simulink model "PSO_PI_Controlled_Booster"  (R2024a)
settings: Solver=VariableStepAuto  StartTime=0.0  StopTime=.2  RelTol=1e-3
values from neighbouring files (symbols this model uses):
  C = 470e-6    (= 0.00047)    [RLC_finder.m]
  Ki = Ki_all(ord(1))    [Run_PI_Optimization.m]    (also in Run_PI_Optimization_paper.m)
  Kp = Kp_all(ord(1))    [Run_PI_Optimization.m]    (also in Run_PI_Optimization_paper.m)
  L = 22.5e-6    (= 2.25e-05)    [RLC_finder.m]    (also in Run_HW_Retest.m = splitlines(string(buf(1:k))))
  R = [2.14277391959 2.34771272008 1.46812094374 4.89216556437 2.35316546958 2.56535436443 0.77405330334 3.72503810805 4.86011715115 3.56120795578 1.74145267632 2.12675435861 ... (240 elements, 8x5x6)]    [HW_Retest.mat]    (also in RLC_finder.m = 50; Run_HW_Retest.m = nan(nD, cfg.nRep, 6); Run_PI_Optimization.m = [Z;Cc]; Run_PI_Optimization_paper.m = [Z;Cc])
  RL = 0.1    [RLC_finder.m]
  Vin = 10    [RLC_finder.m]
  Vout = Vin/(1-D)    (= 18.1818181818)    [RLC_finder.m]
libraries: spsSeriesRLCBranchLib x3, spsCurrentMeasurementLib x2, spsVoltageMeasurementLib x2, spsDCVoltageSourceLib x1, spsDiodeLib x1, spsIGBTLib x1, slpidlib x1, spsPWMGeneratorDCDCLib x1, sps_lib x1
settings Model: Creator=Razowan  LastModifiedBy=Razowan

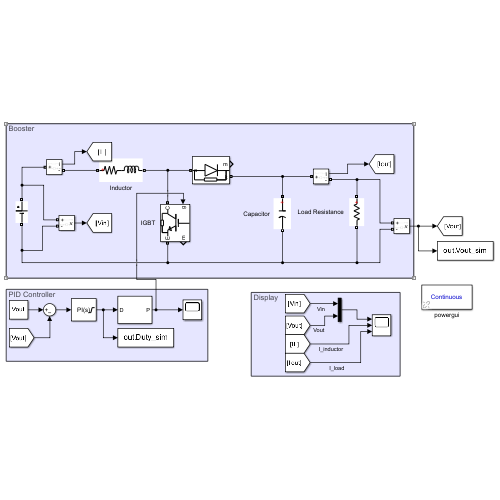
[thumbnail: Simulink's stored preview of the top-level diagram]
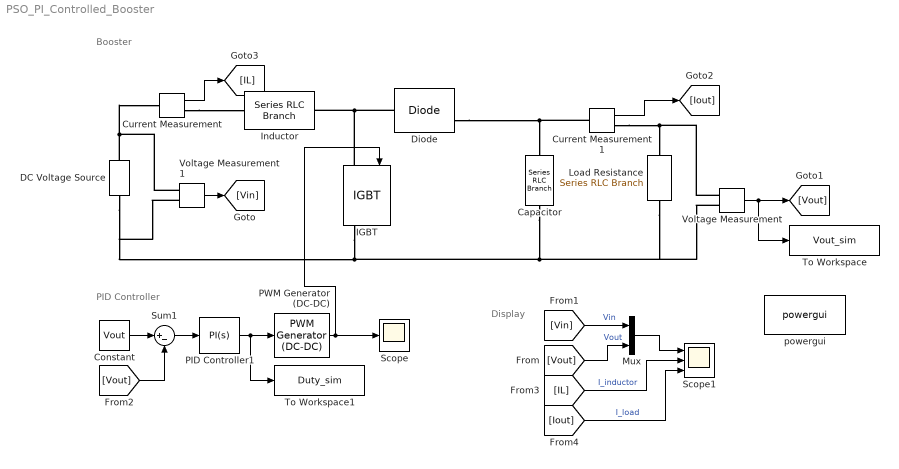
== system PSO_PI_Controlled_Booster ==
  note: Booster
  note: Display
  note: PID Controller
  Capacitor : spsSeriesRLCBranchLib/Series RLC Branch  LConnTagsString=__new0  RConnTagsString=__new0  BranchType=C  Resistance=1  Inductance=L  SetiL0=off  InitialCurrent=0  Capacitance=C  Setx0=off  InitialVoltage=Vin_sim  Measurements=None
  Constant : Constant  Value=Vout
  Current Measurement : spsCurrentMeasurementLib/Current Measurement  PhasorSimulation=off  OutputType=Complex  PSBequivalent=0
  Current Measurement1 : spsCurrentMeasurementLib/Current Measurement  PhasorSimulation=off  OutputType=Complex  PSBequivalent=0
  DC Voltage Source : spsDCVoltageSourceLib/DC Voltage Source  Amplitude=Vin  Measurements=None
  Diode : spsDiodeLib/Diode  Ron=0.001  Lon=0  Vf=0.8  IC=0  UseSnubber=0  Rs=500  Cs=250e-9  Measurements=on
  "IGBT " : spsIGBTLib/IGBT  Ron=0.001  Lon=0  Vf=1  Tf=1e-6  Tt=2e-6  IC=0  Rs=1e5  Cs=inf  Measurements=on
  Inductor : spsSeriesRLCBranchLib/Series RLC Branch  LConnTagsString=__new0  RConnTagsString=__new0  BranchType=RL  Resistance=RL  Inductance=L  SetiL0=off  InitialCurrent=0  Capacitance=1e-6  Setx0=off  InitialVoltage=0  Measurements=None
  "Load Resistance " : spsSeriesRLCBranchLib/Series RLC Branch  LConnTagsString=__new0  RConnTagsString=__new0  BranchType=R  Resistance=R  Inductance=L  SetiL0=off  InitialCurrent=0  Capacitance=1e-6  Setx0=off  InitialVoltage=0  Measurements=None
  Mux : Mux  Inputs=2
  PID Controller1 : slpidlib/PID Controller  Controller=PI  Form=Parallel  TimeDomain=Continuous-time  UseExternalTs=off  SampleTime=-1  IntegratorMethod=Forward Euler  FilterMethod=Forward Euler  ControllerParametersSource=internal  P=Kp  I=Ki  UseKiTs=off  D=0  UseExternalDerivativeSource=off  N=100  UseFilter=on  TunerSelectOption=Transfer Function Based (PID Tuner App)  InitialConditionSource=internal  InitialConditionForIntegrator=0  InitialConditionForFilter=0  DifferentiatorICPrevScaledInput=0  ExternalReset=none  TrackingMode=off  Kt=1  LimitOutput=on  SatLimitsSource=internal  UpperSaturationLimit=0.9  LowerSaturationLimit=0  LinearizeAsGain=on  AntiWindupMode=clamping  Kb=1  LimitIntegrator=off  UpperIntegratorSaturationLimit=inf  LowerIntegratorSaturationLimit=-inf  POutMin=[]  POutMax=[]  IOutMin=[]  IOutMax=[]  DOutMin=[]  DOutMax=[]  NOutMin=[]  NOutMax=[]  SumOutMin=[]  SumOutMax=[]  SaturationOutMin=[]  SaturationOutMax=[]  PParamMin=[]  PParamMax=[]  IParamMin=[]  IParamMax=[]  DParamMin=[]  DParamMax=[]  NParamMin=[]  NParamMax=[]  KbParamMin=[]  KbParamMax=[]  KtParamMin=[]  KtParamMax=[]  KbOutMin=[]  KbOutMax=[]  KtOutMin=[]  KtOutMax=[]  IntegratorOutMin=[]  IntegratorOutMax=[]  FilterOutMin=[]  FilterOutMax=[]  SumI1OutMin=[]  SumI1OutMax=[]  SumI2OutMin=[]  SumI2OutMax=[]  SumI3OutMin=[]  SumI3OutMax=[]  SumI4OutMin=[]  SumI4OutMax=[]  SumDOutMin=[]  SumDOutMax=[]  DifferentiatorOutMin=[]  DifferentiatorOutMax=[]  FilterDiffOutCoefMin=[]  FilterDiffOutCoefMax=[]  ReciprocalOutMin=[]  ReciprocalOutMax=[]  SumDenOutMin=[]  SumDenOutMax=[]  SumNumOutMin=[]  SumNumOutMax=[]  DivideOutMin=[]  DivideOutMax=[]  UdiffTsProdOutMin=[]  UdiffTsProdOutMax=[]  NTsProdOutMin=[]  NTsProdOutMax=[]  UintegralTsProdOutMin=[]  UintegralTsProdOutMax=[]  UngainTsProdOutMin=[]  UngainTsProdOutMax=[]  ClampingZeroOutDataTypeStr=Inherit: Inherit via back propagation  ClampingZeroOutMin=[]  ClampingZeroOutMax=[]  FilterDenConstantOutDataTypeStr=Inherit: Inherit via back propagation  FilterDenConstantOutMin=[]  FilterDenConstantOutMax=[]  PCopyOutDataTypeStr=Inherit: Inherit via back propagation  PCopyOutMin=[]  PCopyOutMax=[]  NCopyOutDataTypeStr=Inherit: Inherit via back propagation  NCopyOutMin=[]  NCopyOutMax=[]  IntegratorContinuousStateAttributes=''  IntegratorStateMustResolveToSignalObject=off  IntegratorRTWStateStorageClass=Auto  FilterContinuousStateAttributes=''  FilterStateMustResolveToSignalObject=off  FilterRTWStateStorageClass=Auto  ParallelPVariant=InternalParameters  IdealPVariant=Disabled  IVariant=InternalParameters  DVariant=Disabled  IntegratorVariant=Continuous  SatVariant=Enabled  AWVariant=ContClampingParallel  PCopyVariant=Disabled  TRVariant=Disabled  FdbkBlocksVariant=Forward  IdealPFdbkVariant=Disabled  SatFdbkVariant=Disabled  DerivativeFilterVariant=Disabled  NVariant=Disabled  NCopyVariant=Disabled_SignalSpec  FilterICVariant=Disabled  IntegratorICVariant=InternalICs  ExternalResetVariant=Disabled  TRSumVariant=Passthrough  SumFdbkVariant=Disabled  SumVariant=Sum_PI  TsampFilterVariant=InternalTs  TsampNgainVariant=Passthrough  TsampIntegralVariant=Disabled_SignalSpec  ExternalSaturationOutDataTypeStr=Inherit: Same as second input  DerivativeSourceVariant=Disabled
  PWM Generator (DC-DC) : spsPWMGeneratorDCDCLib/PWM Generator (DC-DC)  Fsw=fs  Ts=0
  Scope : Scope
  Scope1 : Scope  NumInputPorts=3
  Sum1 : Sum  Inputs=|+-
  To Workspace : ToWorkspace  VariableName=Vout_sim  SaveFormat=Timeseries  SampleTime=-1
  To Workspace1 : ToWorkspace  VariableName=Duty_sim  SaveFormat=Timeseries  SampleTime=-1
  Voltage Measurement : spsVoltageMeasurementLib/Voltage Measurement  PhasorSimulation=off  OutputType=Complex  PSBequivalent=0
  Voltage Measurement1 : spsVoltageMeasurementLib/Voltage Measurement  PhasorSimulation=off  OutputType=Complex  PSBequivalent=0
  powergui : sps_lib/powergui  Priority=1  SimulationMode=Continuous  SampleTime=1e-6  frequency=60  Iterations=50  frequencyindice=0  Pbase=100e6  ErrMax=1e-4  UnitsV=kV  UnitsW=MW  buscounter=0  FunctionMessages=off  echomessages=off  EnableUseOfTLC=off  CurrentSourceSwitches=off  DisableSnubberDevices=off  DisableRonSwitches=off  DisableVfSwitches=off  DisplayEquations=off  AutomaticDiscreteSolvers=off  SolverType=Tustin/Backward Euler (TBE)  Interpol=off  ExternalGateDelay=off  methode=off  Ts=100  x0status=blocks  SPID=on  SwTol=0  HookPort=off  NonlinearTolerance=1e-4  nMaxIteration=100  ContinueOnMaxIteration=off  RestoreLinks=warning  ResistiveCurrentMeasurement=off  Frange=[0:2:500]  Ylog=off  Xlog=on  ShowGrid=off  save=off  variable=ZData  structure=0  ZoomFFT=off  StartTime=0.0  cycles=1  DisplayStyle=1  fundamental=60  FreqAxis=off  MaxFrequency=1000  frequencyindicesteady=1  RmsSteady=1  display=off
  wires:
  Voltage Measurement1/1 -> [Vin]
  Current Measurement/1 -> [IL]
  Current Measurement1/1 -> [Iout]
  PID Controller1/1 -> To Workspace1/1, PWM Generator (DC-DC)/1
  PWM Generator (DC-DC)/1 -> Scope/1, "IGBT "/1
  Sum1/1 -> PID Controller1/1
  Constant/1 -> Sum1/1
  [Vout] -> Sum1/2
  Voltage Measurement/1 -> To Workspace/1, [Vout]
  Mux/1 -> Scope1/1
  [Vin] -> Mux/1  "Vin"
  [Vout] -> Mux/2  "Vout"
  [IL] -> Scope1/2  "I_inductor"
  [Iout] -> Scope1/3  "I_load"
  connections:
  Current Measurement/RConn1 -- Inductor/LConn1
  Voltage Measurement1/LConn1 -- DC Voltage Source/RConn1 -- Current Measurement/LConn1
  Diode/LConn1 -- "IGBT "/LConn1 -- Inductor/RConn1
  "IGBT "/RConn1 -- DC Voltage Source/LConn1 -- Voltage Measurement1/LConn2 -- Capacitor/RConn1 -- Voltage Measurement/LConn2 -- "Load Resistance "/RConn1
  Diode/RConn1 -- Current Measurement1/LConn1 -- Capacitor/LConn1
  Voltage Measurement/LConn1 -- Current Measurement1/RConn1 -- "Load Resistance "/LConn1
